simulink model "Powertrain"  (R2026a)
settings: Solver=FixedStepAuto  StopTime=1372  FixedStep=0.5
values from neighbouring files (symbols this model uses):
  Cd = 0.28    [Imports.m]    (also in Imports_2GR.m; TWOSPEED_TRANS_OPTI.m; gr_SIZING_IMPORTS.m)
  Crf = 0.015    [Imports.m]    (also in Imports_2GR.m; TWOSPEED_TRANS_OPTI.m; gr_SIZING_IMPORTS.m)
  Fa = 3.8056    [Imports.m]    (also in Imports_2GR.m; TWOSPEED_TRANS_OPTI.m; gr_SIZING_IMPORTS.m)
  GR = 7.96    [Imports.m]    (also in gr_SIZING_IMPORTS.m = GR_set(i))
  GVM = Mv + Md    (= 1710.665)    [Imports.m]    (also in Imports_2GR.m = 1730.665; TWOSPEED_TRANS_OPTI.m = 1730.665; gr_SIZING_IMPORTS.m)
  GVW = GVM*g    (= 16781.62365)    [Imports.m]    (also in Imports_2GR.m = 16977.82365; TWOSPEED_TRANS_OPTI.m = 16977.82365; gr_SIZING_IMPORTS.m)
  Meff_eff = Meff(:,2:16)    [Imports.m]    (also in Imports_2GR.m; TWOSPEED_TRANS_OPTI.m; gr_SIZING_IMPORTS.m; gr_SIZING_IMPORTS_2R.m)
  Meff_Speed = Meff(:,1)    [Imports.m]    (also in Imports_2GR.m; TWOSPEED_TRANS_OPTI.m; gr_SIZING_IMPORTS.m; gr_SIZING_IMPORTS_2R.m)
  Meff_Torque = Meff(:,17)    [Imports.m]    (also in Imports_2GR.m; TWOSPEED_TRANS_OPTI.m; gr_SIZING_IMPORTS.m = Meff(1:size(Meff_eff,2), 17); gr_SIZING_IMPORTS_2R.m = Meff(1:size(Meff_eff,2), 17))
  rho = 1.225    [Imports.m]    (also in Imports_2GR.m; TWOSPEED_TRANS_OPTI.m; gr_SIZING_IMPORTS.m)
  Rw = 0.2032    [Imports.m]    (also in Imports_2GR.m; TWOSPEED_TRANS_OPTI.m; gr_SIZING_IMPORTS.m)
  Teff = 0.89    [Imports.m]    (also in Imports_2GR.m; TWOSPEED_TRANS_OPTI.m; gr_SIZING_IMPORTS.m)
settings Model: Creator=goodbox  LastModifiedBy=sujee

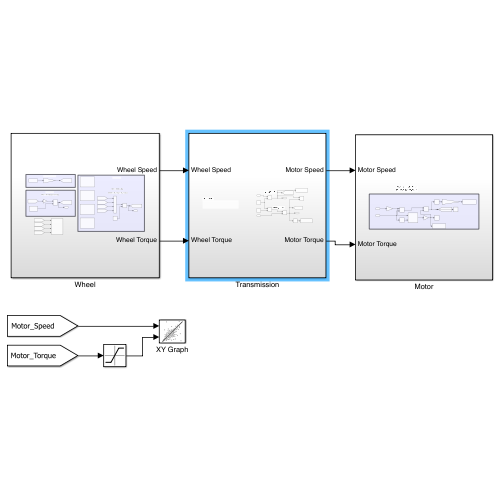
[thumbnail: Simulink's stored preview of the top-level diagram]
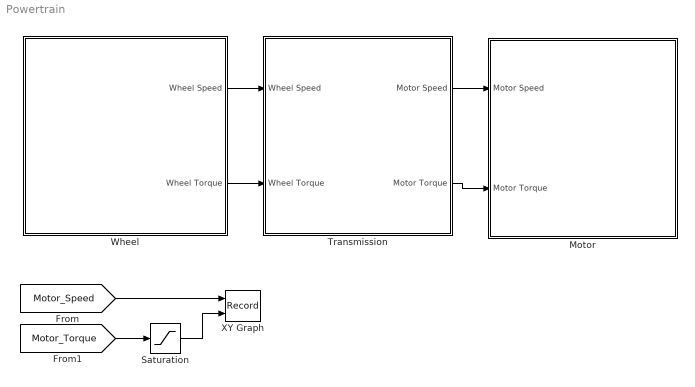
== system Powertrain ==
  Motor : Subsystem
  Saturation : Saturate  UpperLimit=inf  LowerLimit=0
  Transmission : Subsystem
  Wheel : Subsystem
  XY Graph : Record  NumPorts=2.0  FileSettingsInternal="{\"entries\":[{\"content\":{\"excelSettings\":{\"content\":{},\"type\":\"Streamout.ExcelSettings\"},\"parquetSettings\":{\"content\":{},\"type\":\"Streamout.ParquetSettings\"}},\"type\":\"Streamout.FileSettingStorage\",\"uuid\":\"\"}],\"packageUris\":[\"http:\\/\\/schema.mathworks.com\\/mf0\\/streamout_blocks\\/R2020a\"],\"version\":\"1.0\"}"  FrameSettings=[0, 0]  Layout=[1 1]  SignalsInternal="{\"entries\":[{\"content\":{\"signals\":[{\"content\":{\"blockPath\":[],\"dimensions\":[1],\"domain\":\"\",\"lineColor\":\"#a2142f\",\"plots\":[ 1 ],\"port\":1,\"sid\":[\"\"],\"signalID\":1,\"signalName\":\"From\"},\"type\":\"RecordBlkView.Signal\",\"uuid\":\"\"},{\"content\":{\"blockPath\":[],\"dimensions\":[1],\"domain\":\"\",\"lineColor\":\"#139fff\",\"plots\":[ 1 ],\"port\":2,\"sid\":[\"\"],\"signalID\":2,\"signalName\":\"Saturation\"},\"type\":\"RecordBlkView.Signal\",\"uuid\":\"\"}]},\"type\":\"RecordBlkView.InputSignals\",\"uuid\":\"\"}],\"packageUris\":[\"http:\\/\\/schema.mathworks.com\\/mf0\\/streamout_blocks\\/R2020a\"],\"version\":\"1.0\"}"  VisualizationBindings="{\"xyplotplugin\":{\"info\":[{\"series\":[{\"bindingParametersList\":[{\"parameter\":\"X-Axis\",\"signalID\":1,\"signalName\":\"From\"},{\"parameter\":\"Y-Axis\",\"signalID\":2,\"signalName\":\"Saturation\"}],\"seriesID\":0}],\"subplotID\":1}]}}"  CompatibilityTag=XY
  wires:
  Wheel/1(Wheel Speed) -> Transmission/1(Wheel Speed)
  Wheel/2(Wheel Torque) -> Transmission/2(Wheel Torque)
  Transmission/1(Motor Speed) -> Motor/1(Motor Speed)
  Transmission/2(Motor Torque) -> Motor/2(Motor Torque)
  [Motor_Speed] -> XY Graph/1
  [Motor_Torque] -> Saturation/1
  Saturation/1 -> XY Graph/2

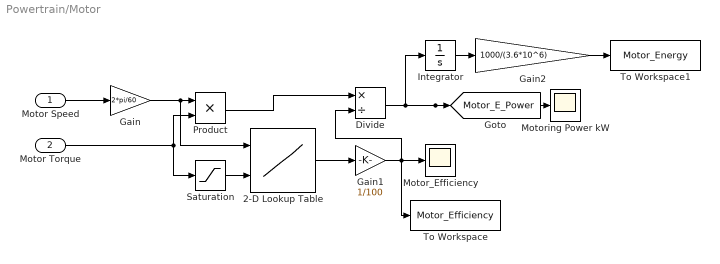
== system Powertrain/Motor ==
  Motor Speed : Inport
  Motor Torque : Inport  Port=2
  2-D Lookup Table : Lookup_n-D  BreakpointsForDimension1=Meff_Speed  BreakpointsForDimension2=Meff_Torque  Table=Meff_eff  InternalRulePriority=Speed  RndMeth=Simplest
      settings: InputPortMap=u0,u1
  Divide : Product  Inputs=*/
  Gain : Gain  Gain=2*pi/60
  Gain1 : Gain  Gain=1/100
  Gain2 : Gain  Gain=1000/(3.6*10^6)
  Integrator : Integrator
  Motor_Efficiency : Scope
      settings: ActiveDisplayYMinimum=-1  ActiveDisplayYMaximum=1  DataLoggingVariableName=ScopeData3
  Motoring Power kW : Scope
      settings: ActiveDisplayYMinimum=-1  ActiveDisplayYMaximum=1  DataLoggingVariableName=ScopeData4
  Product : Product
  Saturation : Saturate  UpperLimit=inf  LowerLimit=0
  To Workspace : ToWorkspace  VariableName=Motor_Efficiency  SaveFormat=Timeseries  SampleTime=-1
  To Workspace1 : ToWorkspace  VariableName=Motor_Energy  SaveFormat=Timeseries  SampleTime=-1
  tag scope: Motor_E_Power=global
  wires:
  Motor Speed/1 -> Gain/1
  Gain/1 -> 2-D Lookup Table/1, Product/1
  Motor Torque/1 -> Product/2, Saturation/1
  2-D Lookup Table/1 -> Gain1/1
  Product/1 -> Divide/1
  Gain1/1 -> To Workspace/1, Divide/2, Motor_Efficiency/1
  Saturation/1 -> 2-D Lookup Table/2
  Divide/1 -> Integrator/1, [Motor_E_Power], Motoring Power kW/1
  Integrator/1 -> Gain2/1
  Gain2/1 -> To Workspace1/1

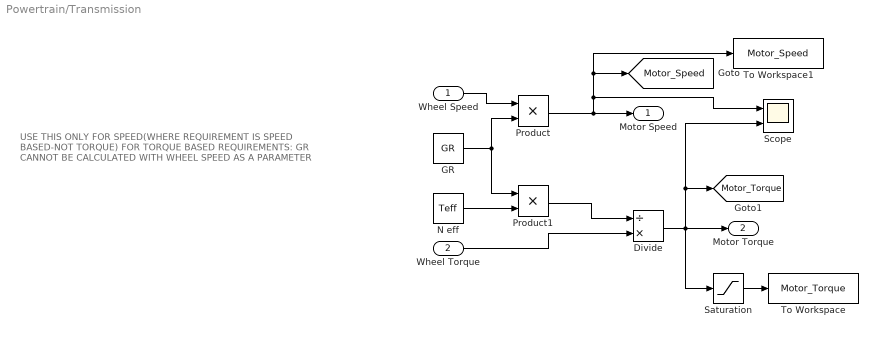
== system Powertrain/Transmission ==
  note: USE THIS ONLY FOR SPEED(WHERE REQUIREMENT
      | IS SPEED BASED-NOT TORQUE)
      |
      | FOR TORQUE BASED REQUIREMENTS: GR CANNOT BE
      | CALCULATED WITH WHEEL SPEED AS A PARAMETER
  Wheel Speed : Inport
  Wheel Torque : Inport  Port=2
  Divide : Product  Inputs=/*
  GR : Constant  Value=GR
  N eff : Constant  Value=Teff
  Product : Product
  Product1 : Product
  Saturation : Saturate  UpperLimit=inf  LowerLimit=0
  Scope : Scope  NumInputPorts=2
      settings: ActiveDisplayYMinimum=-1185.22041  ActiveDisplayYMaximum=10666.98373
  To Workspace : ToWorkspace  VariableName=Motor_Torque  SaveFormat=Timeseries  SampleTime=-1
  To Workspace1 : ToWorkspace  VariableName=Motor_Speed  SaveFormat=Timeseries  SampleTime=-1
  Motor Speed : Outport
  Motor Torque : Outport  Port=2
  tag scope: Motor_Speed=global, Motor_Torque=global
  wires:
  Wheel Speed/1 -> Product/1
  GR/1 -> Product1/1, Product/2
  N eff/1 -> Product1/2
  Product1/1 -> Divide/1
  Wheel Torque/1 -> Divide/2
  Product/1 -> To Workspace1/1, [Motor_Speed], Scope/1, Motor Speed/1
  Divide/1 -> Saturation/1, Scope/2, [Motor_Torque], Motor Torque/1
  Saturation/1 -> To Workspace/1

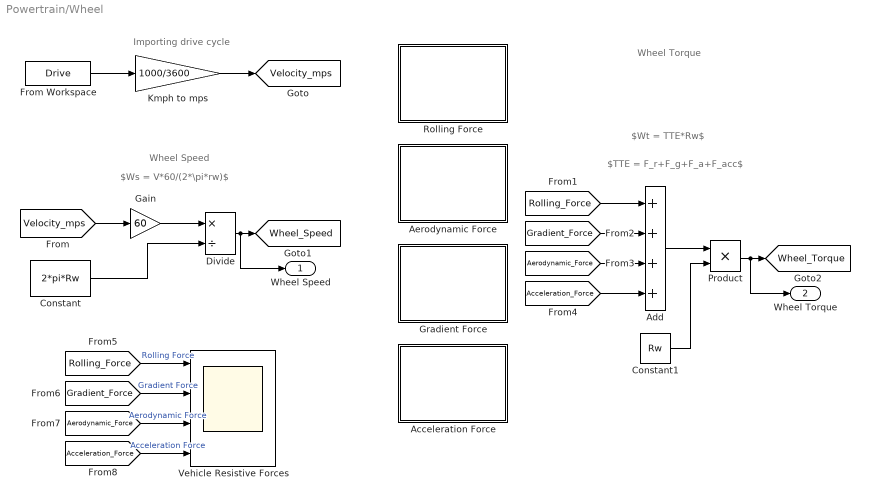
== system Powertrain/Wheel ==
  note: $TTE = F_r+F_g+F_a+F_acc$
  note: $Wt = TTE*Rw$
  note: Wheel Torque
  note: $Ws = V*60/(2*\pi*rw)$
  note: Wheel Speed
  note: Importing drive cycle
  Acceleration Force : Subsystem
  Add : Sum  Inputs=4
  Aerodynamic Force : Subsystem
  Constant : Constant  Value=2*pi*Rw
  Constant1 : Constant  Value=Rw
  Divide : Product  Inputs=*/
  From Workspace : FromWorkspace  VariableName=Drive
  Gain : Gain  Gain=60
  Gradient Force : Subsystem
  Kmph to mps : Gain  Gain=1000/3600
  Product : Product
  Rolling Force : Subsystem
  Vehicle Resistive Forces : Scope  NumInputPorts=4
      settings: ActiveDisplayYMinimum=151.72435475  ActiveDisplayYMaximum=351.72435475
  Wheel Speed : Outport
  Wheel Torque : Outport  Port=2
  tag scope: Velocity_mps=global, Wheel_Speed=global, Wheel_Torque=global
  wires:
  From Workspace/1 -> Kmph to mps/1
  Kmph to mps/1 -> [Velocity_mps]
  [Velocity_mps] -> Gain/1
  Gain/1 -> Divide/1
  Constant/1 -> Divide/2
  Divide/1 -> Wheel Speed/1, [Wheel_Speed]
  [Rolling_Force] -> Add/1
  [Gradient_Force] -> Add/2
  [Aerodynamic_Force] -> Add/3
  [Acceleration_Force] -> Add/4
  Add/1 -> Product/1
  Constant1/1 -> Product/2
  Product/1 -> Wheel Torque/1, [Wheel_Torque]
  [Rolling_Force] -> Vehicle Resistive Forces/1  "Rolling Force"
  [Gradient_Force] -> Vehicle Resistive Forces/2  "Gradient Force"
  [Aerodynamic_Force] -> Vehicle Resistive Forces/3  "Aerodynamic Force"
  [Acceleration_Force] -> Vehicle Resistive Forces/4  "Acceleration Force"

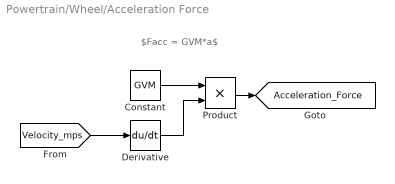
== system Powertrain/Wheel/Acceleration Force ==
  note: $Facc = GVM*a$
  Constant : Constant  Value=GVM
  Derivative : Derivative
  Product : Product
  tag scope: Acceleration_Force=global
  wires:
  [Velocity_mps] -> Derivative/1
  Constant/1 -> Product/1
  Derivative/1 -> Product/2
  Product/1 -> [Acceleration_Force]

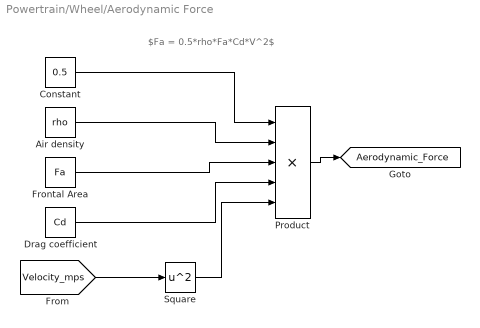
== system Powertrain/Wheel/Aerodynamic Force ==
  note: $Fa = 0.5*rho*Fa*Cd*V^2$
  Air density : Constant  Value=rho
  Constant : Constant  Value=0.5
  Drag coefficient : Constant  Value=Cd
  Frontal Area : Constant  Value=Fa
  Product : Product  Inputs=5
  Square : Math  Operator=square
  tag scope: Aerodynamic_Force=global
  wires:
  [Velocity_mps] -> Square/1
  Square/1 -> Product/5
  Drag coefficient/1 -> Product/4
  Frontal Area/1 -> Product/3
  Air density/1 -> Product/2
  Constant/1 -> Product/1
  Product/1 -> [Aerodynamic_Force]

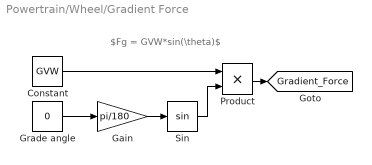
== system Powertrain/Wheel/Gradient Force ==
  note: $Fg = GVW*sin(\theta)$
  Constant : Constant  Value=GVW
  Gain : Gain  Gain=pi/180
  Grade angle : Constant  Value=0
  Product : Product
  Sin : Trigonometry
  tag scope: Gradient_Force=global
  wires:
  Grade angle/1 -> Gain/1
  Gain/1 -> Sin/1
  Constant/1 -> Product/1
  Sin/1 -> Product/2
  Product/1 -> [Gradient_Force]

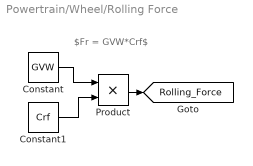
== system Powertrain/Wheel/Rolling Force ==
  note: $Fr = GVW*Crf$
  Constant : Constant  Value=GVW
  Constant1 : Constant  Value=Crf
  Product : Product
  tag scope: Rolling_Force=global
  wires:
  Constant/1 -> Product/1
  Constant1/1 -> Product/2
  Product/1 -> [Rolling_Force]
